simulink model "main"  (R2026b)
settings: Solver=ode45  StopTime=30  MaxStep=0.01  RelTol=1e-6  AbsTol=1e-8
PostLoadFcn:
  | run(fullfile(fileparts(get_param(bdroot,'FileName')),'Pendulo_Invertido.m'));
values from neighbouring files (symbols this model uses):
  Kd_theta = 2*zeta_theta*omega_theta    (= 19.6)    [Pendulo_Invertido.m]
  Kdx = 2*zeta_x*omega_x/g    (= 0.183548918336)    [Pendulo_Invertido.m]
  Ki_theta = 0    [Pendulo_Invertido.m]
  Kix = 0    [Pendulo_Invertido.m]
  Kp_theta = omega_theta^2    (= 196)    [Pendulo_Invertido.m]
  Kpx = omega_x^2/g    (= 0.101971621298)    [Pendulo_Invertido.m]
settings Model: Creator=fedeb  LastModifiedBy=fedeb
settings SolverCC: MaxConsecutiveMinStep=5
settings SimscapeCC: SimscapeLogType=all  SimscapeNominalValues="[{\"value\":\"1\",\"unit\":\"A\"},{\"value\":\"1\",\"unit\":\"bar\"},{\"value\":\"1\",\"unit\":\"cm^2\"},{\"value\":\"1\",\"unit\":\"cm^3/s\"},{\"value\":\"1\",\"unit\":\"kJ/kg\"},{\"value\":\"1\",\"unit\":\"kW\"},{\"value\":\"1\",\"unit\":\"l\"},{\"value\":\"1\",\"unit\":\"N\"},{\"value\":\"1\",\"unit\":\"N*m\"},{\"value\":\"1\",\"unit\":\"V\"},{\"value\":\"0.001\",\"unit\":\"Wb\"}]"  SimscapeUseEnergyAccounting=off

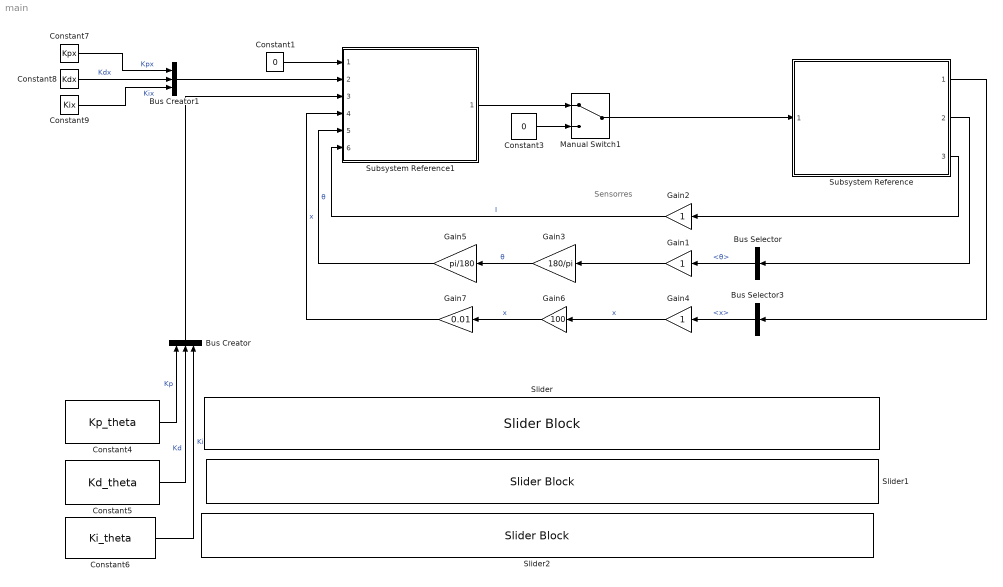
== system main ==
  note: Sensorres
  Bus Creator : BusCreator  Inputs=3
  Bus Creator1 : BusCreator  Inputs=3
  Bus Selector : BusSelector  OutputSignals=θ
  Bus Selector3 : BusSelector  OutputSignals=x
  Constant1 : Constant  Value=0
  Constant3 : Constant  Value=0
  Constant4 : Constant  Value=Kp_theta
  Constant5 : Constant  Value=Kd_theta
  Constant6 : Constant  Value=Ki_theta
  Constant7 : Constant  Value=Kpx
  Constant8 : Constant  Value=Kdx
  Constant9 : Constant  Value=Kix
  Gain1 : Gain
  Gain2 : Gain
  Gain3 : Gain  Gain=180/pi
  Gain4 : Gain
  Gain5 : Gain  Gain=pi/180
  Gain6 : Gain  Gain=100
  Gain7 : Gain  Gain=0.01
  Manual Switch1 : ManualSwitch
  Slider : SliderBlock  ScaleMax=50
  Slider1 : SliderBlock  ScaleMax=20
  Slider2 : SliderBlock  ScaleMax=5
  Subsystem Reference : Subsystem  ReferencedSubsystem=Planta
  Subsystem Reference1 : Subsystem  ReferencedSubsystem=Controlador
  wires:
  Constant1/1 -> Subsystem Reference1/1
  Bus Selector/1 -> Gain1/1  "<θ>"
  Bus Selector3/1 -> Gain4/1  "<x>"
  Constant5/1 -> Bus Creator/2  "Kd"
  Constant4/1 -> Bus Creator/1  "Kp"
  Constant6/1 -> Bus Creator/3  "Ki"
  Bus Creator/1 -> Subsystem Reference1/3
  Bus Creator1/1 -> Subsystem Reference1/2
  Constant8/1 -> Bus Creator1/2  "Kdx"
  Constant7/1 -> Bus Creator1/1  "Kpx"
  Constant9/1 -> Bus Creator1/3  "Kix"
  Subsystem Reference1/1 -> Manual Switch1/1
  Constant3/1 -> Manual Switch1/2
  Subsystem Reference/2 -> Bus Selector/1
  Subsystem Reference/1 -> Bus Selector3/1
  Gain1/1 -> Gain3/1
  Manual Switch1/1 -> Subsystem Reference/1
  Gain4/1 -> Gain6/1  "x"
  Gain3/1 -> Gain5/1  "θ"
  Gain5/1 -> Subsystem Reference1/5  "θ"
  Subsystem Reference/3 -> Gain2/1
  Gain2/1 -> Subsystem Reference1/6  "Ⅰ"
  Gain6/1 -> Gain7/1  "x"
  Gain7/1 -> Subsystem Reference1/4  "x"
